simulink library "roblocks"  (R2019a)
settings: Solver=ode45  StartTime=0.0  StopTime=10  RelTol=1e-3  EnableMultiTasking=on
values from neighbouring files (symbols this model uses):
  q = 1    [quadrotor_plot.m]
undefined symbols (not defined in the file or in its folder): a, angdiff, camera, cinertia, cond, delta2tr, eul2tr, fkine, gravload, inertia, jacob0, jacobe, numcols, P, p560, purepursuit, qd, qdd, qz, rne, robot, rpy2tr, tr2delta, tr2eul, tr2rpy, transl, trnorm, trotz, v_max
(part 1 of 2)
settings Model: Creator=n6334687  LastModifiedBy=corkep
settings DataIOCC: LimitDataPoints=on  SaveFormat=Array  SignalLoggingSaveFormat=ModelDataLogs  ReturnWorkspaceOutputs=off
settings OptimizationCC: ExpressionDepthLimit=2147483647  LifeSpan=inf
settings DebuggingCC: UnderspecifiedInitializationDetection=Classic  MergeDetectMultiDrivingBlocksExec=none  SolverPrmCheckMsg=warning  FcnCallInpInsideContextMsg=warning  AllowSymbolicDim=off  StateNameClashWarn=warning  PregeneratedLibrarySubsystemCodeDiagnostic=none  SFUnexpectedBacktrackingDiag=warning  SFNoUnconditionalDefaultTransitionDiag=warning  SFExecutionAtInitializationDiag=none  ArithmeticOperatorsInVariantConditions=warning
settings HardwareCC: ProdBitPerPointer=32  ProdBitPerSizeT=32  ProdBitPerPtrDiffT=32  ProdLargestAtomicFloat=None  ProdIntDivRoundTo=Undefined  ProdEndianess=Unspecified  ProdWordSize=32  ProdHWDeviceType=32-bit Generic
settings ModelReferenceCC: PropagateSignalLabelsOutOfModel=off
settings SFSimCC: SimUseLocalCustomCode=off
settings RTWCC: RTWUseLocalCustomCode=off
settings CodeAppCC: StateflowObjectComments=on
settings GRTTargetCC: TargetLangStandard=C89/C90 (ANSI)  GeneratePreprocessorConditionals=Disable all  CombineOutputUpdateFcns=off  GRTInterface=on
settings ConfigComp: CovMetricSettings=dw  CovHtmlReporting=on  CovSaveCumulativeToWorkspaceVar=on  CovSaveSingleToWorkspaceVar=on  CovExternalEMLEnable=off  CovSFcnEnable=off

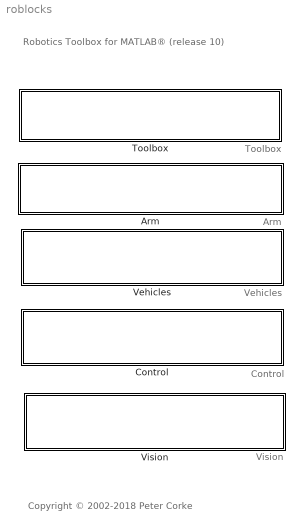
== system roblocks ==
  note: Vision
  note: Control
  note: Vehicles
  note: Arm
  note: Toolbox
  note: Robotics Toolbox for MATLAB®
      | (release 10)
  note: Copyright © 2002-2018 Peter Corke
  Arm : Subsystem
      mask Display: disp('Robot arms')
  Control : Subsystem
      mask Display: disp('Control')
  Toolbox : Subsystem
      mask Display: disp('Toolbox functions')
  Vehicles : Subsystem
      mask Display: disp('Vehicles: wheeled, flying')
  Vision : Subsystem
      mask Display: disp('Vision')

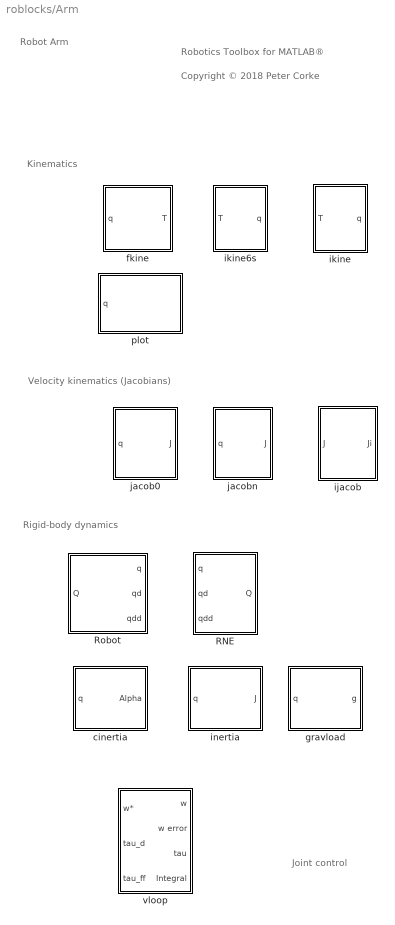
== system roblocks/Arm ==
  note: Robot
      | Arm
  note: Kinematics
  note: Velocity kinematics (Jacobians)
  note: Rigid-body dynamics
  note: Joint control
  note: Copyright © 2018 Peter Corke
  note: Robotics Toolbox for MATLAB®
  RNE : Subsystem  mask{robot=robot, grav=[0 0 9.81]}
      mask prompts: robot "Robot object"; grav "Gravity"
      mask help: Rigid-body inverse dynamics.
      mask init:
      | if isa(robot, 'SerialLink')
      |     n = robot.n
      |     rname = robot.name;
      | else
      |     n = 0;
      |     rname = '';
      | end
      mask Help:
      | Given a robot dynamic model and joint angle, rate and acceleration
      | determine the required joint torque.
      | 
      | <b>Parameters::</b>
      | 
      | robot (SerialLink) a dynamic model of an N-link serial link manipulator
      | gravity (1x3)  IGNORED Gravitational acceleration in world frame [m/s2]
      | 
      | <b>Inputs::</b>
      | 
      | q (1xN) joint coordinates
      | qd (1xN) joint coordinate velocity
      | qdd (1xN) joint coordinate acceleration
      | 
      | 
      | <b>Outputs::</b>
      | 
      | Q (1xN) the generalized joint force (torque or force) required to achieve
      | the motion state (q, qd, qdd).
      | 
      | <b>Notes::</b>
      | 
      | - Required for computed and inverse torque control schemes.
      | - The gravity parameter is ignored.
      | - Implemented using the recursive Newton-Euler scheme (RNE).
      | - A wrapper for the Toolbox method rne().
      mask Display:
      | port_label('output', 1, 'Q')
      | port_label('input', 1, 'q')
      | port_label('input', 2, 'qd')
      | port_label('input', 3, 'qdd')
      | text(0.9, 0.9,  rname, 'horizontalAlignment', 'right')
  Robot : Subsystem  mask{robot=robot, q0=[0 0 0 0 0 0]}
      mask prompts: robot "Robot object"; q0 "Initial state"
      mask help: Rigid-body dynamic model of robot.
      mask init:
      | if isa(robot, 'SerialLink')
      |     rname = robot.name;
      |     %fprintf('**robot name is %s\n', rname);
      | else
      |     rname = '';
      |     n = 0
      | end
      mask Help:
      | Simulates the forward (direct) rigid-body dynamics of the robot described
      | by the given robot object.  For given applied joint torque/force it computes
      | the instaneous joint coordinates, velocities and acclerations.
      | 
      | 
      | <b>Parameters::</b>
      | 
      | robot (SerialLink) a dynamic model of an N-link serial link manipulator
      | q0 (1xN)  Initial joint coordinates
      | 
      | <b>Inputs::</b>
      | 
      | Q (1xN) the generalized joint force (torque or force) required to achieve
      | the motion state (q, qd, qdd).
      | 
      | <b>Outputs::</b>
      | 
      | q (1xN) joint coordinates
      | qd (1xN) joint coordinate velocity
      | qdd (1xN) joint coordinate acceleration
      | 
      | 
      | <b>Notes::</b>
      | 
      | - Required to simulate robot rigid body motion.
      | - Implemented using the recursive Newton-Euler scheme (RNE).
      | - A wrapper for the Toolbox method accel() which in turn depends on the
      |   method rne().
      mask Display:
      | port_label('input', 1, 'Q')
      | port_label('output', 1, 'q')
      | port_label('output', 2, 'qd')
      | port_label('output', 3, 'qdd')
      | text(0.1, 0.9,  rname, 'horizontalAlignment', 'left')
  cinertia : Subsystem  mask{robot=0}
  fkine : Subsystem  mask{robot=robot}
      mask prompts: robot "Robot object"
      mask help: Robot forward kinematics.
      mask Help:
      | Compute homogeneous transform for robot end-effector given joint coordinates
      | 
      | 
      | <b>Parameters::</b>
      | 
      | Robot (SerialLink class)  The N-axis robot object for computing forward kinematics.
      | 
      | <b>Inputs::</b>
      | 
      | q (1xN) joint coordinates
      | 
      | <b>Outputs::</b>
      | 
      | T (4x4) the pose of the end effector as a homogeneous transformation
      | 
      | <b>Notes::</b>
      | 
      | - A wrapper for the Toolbox method fkine().
      mask Display:
      | port_label('input', 1, 'q')
      | port_label('output', 1, 'T')
      | if ~isempty(robot)
      |     text(0.5, 0.2, robot.name,  'horizontalAlignment', 'center')
      | end
  gravload : Subsystem  mask{robot=0}
  ijacob : Subsystem
      mask help: Inverse Jacobian
      mask Help:
      | Inverse of Jacobian matrix which maps spatial velocity to joint coordinate
      | rates.
      | 
      | 
      | <b>Inputs::</b>
      | 
      | J (6x6) the Jacobian matrix
      | 
      | <b>Outputs::</b>
      | 
      | Ji (6x6) the inverse Jacobian matrix
      | 
      | <b>Notes::</b>
      | 
      | - A wrapper for the MATLAB function inv().
      | - Only valid for square Jacobians (6-axis robots)
      mask Display:
      | text(0.4, 0.7, '\bf\fontsize{16}J', 'texmode', 'on', 'verticalAlignment', 'top', 'horizontalAlignment', 'left')
      | text(0.6, 0.65, '\fontsize{10}-1', 'texmode', 'on','verticalAlignment', 'bottom', 'horizontalAlignment', 'left')
      | port_label('input', 1, 'J');
      | port_label('output', 1, 'Ji')
  ikine : Subsystem  mask{robot=p560, q0=qz, M=[1 1 1 1 1 1], pinv=off, options={}}
      mask prompts: robot "Robot object"; q0 "Initial q"; M "Mask vector"; pinv "Pseudo-inverse (pinv)"; options "Options (cell array)"
      mask help: Generalized numerical inverse kinematics
      mask init:
      | opt = options;
      | if pinv
      |     opt = [opt 'pinv'];
      | end
      | disp(opt)
      mask Help:
      | Compute joint coordinates for robot given end-effector pose.
      | 
      | 
      | <b>Parameters::</b>
      | 
      | Robot (SerialLink class)  The N-axis robot object for computing forward kinematics.
      | Initial q  (1xN)          Initial joint coordinates for solution
      | Mask vector (1x6)         Mask vector for underactuated manipulators.
      | Pseudo inverse (logical)  Enable option 'pinv'
      | Options                   Option value list to be passed to ikine()
      | 
      | <b>Inputs::</b>
      | 
      | T (4x4) the pose of the end effector as a homogeneous transformation
      | 
      | 
      | <b>Outputs::</b>
      | 
      | q (1xN) joint coordinates
      | 
      | <b>Notes::</b>
      | 
      | - A wrapper for the Toolbox method ikine().
  ikine6s : Subsystem  mask{robot=p560, conf='luf'}
      mask prompts: robot "Robot object"; conf "Configuration string"
      mask help: Inverse kinematics for 6-axis spherical robot
      mask Help:
      | Compute joint coordinates for robot given end-effector pose.
      | 
      | 
      | <b>Parameters::</b>
      | 
      | Robot (SerialLink class)  The N-axis robot object for computing forward kinematics.
      | Configuration             Configuration string comprised of 'lrudnf'
      | 
      | <b>Inputs::</b>
      | 
      | T (4x4) the pose of the end effector as a homogeneous transformation
      | 
      | 
      | <b>Outputs::</b>
      | 
      | q (1xN) joint coordinates
      | 
      | <b>Notes::</b>
      | 
      | - A wrapper for the Toolbox method ikine6s().
  inertia : Subsystem  mask{robot=0}
  "jacob0 " : Subsystem  mask{robot=robot}
      mask prompts: robot "Robot object"
      mask help: Robot Jacobian in world coordinates
      mask init:
      | if ~isempty(robot)
      |     n=robot.n;
      | end
      mask Help:
      | Jacobian matrix relating joint coordinate rates to end-effector spatial
      | velocity expressed in the world frame.
      | 
      | <b>Parameters::</b>
      | 
      | Robot (SerialLink class)  The N-axis robot object for which the Jacobian is
      |                           computed.
      | 
      | <b>Inputs::</b>
      | 
      | q (1xN) joint coordinates
      | 
      | <b>Outputs::</b>
      | 
      | J (6xN) the Jacobian matrix
      | 
      | <b>Notes::</b>
      | 
      | - A wrapper for the Toolbox method jacob0().
      mask Display:
      | text(0.4, 0.7, '\bf\fontsize{16}J', 'texmode', 'on', 'verticalAlignment', 'top', 'horizontalAlignment', 'left')
      | text(0.45, 0.65, '\fontsize{10}0', 'texmode', 'on','verticalAlignment', 'bottom', 'horizontalAlignment', 'right')
      | if ~isempty(robot)
      |     text(0.5, 0.2, robot.name,  'horizontalAlignment', 'center')
      | end
      | port_label('input', 1, 'q')
      | port_label('output', 1, 'J')
  jacobn : Subsystem  mask{robot=robot}
      mask prompts: robot "Robot object"
      mask help: Robot Jacobian in end-effector coordinates
      mask init:
      | n=robot.n;
      mask Help:
      | Jacobian matrix relating joint coordinate rates to end-effector spatial
      | velocity expressed in the end-effector frame.
      | 
      | <b>Parameters::</b>
      | 
      | Robot (SerialLink class)  The N-axis robot object for which the Jacobian is
      |                           computed.
      | 
      | <b>Inputs::</b>
      | 
      | q (1xN) joint coordinates
      | 
      | <b>Outputs::</b>
      | 
      | J (6xN) the Jacobian matrix
      | 
      | <b>Notes::</b>
      | 
      | - A wrapper for the Toolbox method jacobn().
      mask Display:
      | text(0.4, 0.7, '\bf\fontsize{16}J', 'texmode', 'on', 'verticalAlignment', 'top', 'horizontalAlignment', 'left')
      | text(0.45, 0.65, '\fontsize{10}N', 'texmode', 'on','verticalAlignment', 'bottom', 'horizontalAlignment', 'right')
      | if ~isempty(robot)
      |     text(0.5, 0.2, robot.name,  'horizontalAlignment', 'center')
      | end
      | port_label('input', 1, 'q')
      | port_label('output', 1, 'J')
  plot : Subsystem  mask{robot=p560, fps=5, holdplot=on}
      mask prompts: robot "Robot object"; fps "Update rate (fps)"; holdplot "Hold"
      mask help: Graphical robot display.
      mask Help:
      | This block graphically displays the passed SerialLink class object.
      | 
      | A new figure is created and the robot is animated (using SerialLink.plot)
      | to a pose specified by the joint coordinate vector input to the block whose
      | width must match the number of robot joints.
      | 
      | If the Hold checkbox is ticked then a "hold" command is issued at initialization
      | time allowing multiple robots to be displayed in the one plot.
      mask Display:
      | port_label('input', 1, 'q')
      | if ~isempty(robot)
      |     text(0.5, 0.2, robot.name,  'horizontalAlignment', 'center')
      | end
  vloop : Subsystem  mask{J=372e-6, B=817e-6, Km=0.228, tau_max=0.9, Kv=1, Ki=0, T=0.001}
      mask prompts: J "Inertia (J)"; B "Viscous friction coefficient (B)"; Km "Motor torque constant"; tau_max "Torque limit (tau_max)"; Kv "Proportional gain (Kv)"; Ki "Integral gain (Ki)"; T "Sample interval (T)"

== system roblocks/Control ==
  note: Robotics Toolbox for MATLAB®
  note: Copyright © 2018 Peter Corke
  note: Control
  note: Motor control
  vloop_voltage : Subsystem  mask{J=372e-6, B=817e-6, Km=0.228, tau_max=20, Rm=0.1, Lm=0.1, Ka=10, Kv=1, Ki=1, T=0.001}
      mask prompts: J "Inertia (K)"; B "Viscous friction coefficient (B)"; Km "Motor torque constant"; tau_max "Voltage limit (tau_max)"; Rm "Motor resistance (Rm)"; Lm "Motor inductance (Lm)"; Ka "Amplifier gain (Ka)"; Kv "Proportional gain (Kv)"; Ki "Integral gain (Ki)"; T "Sample interval (T)"

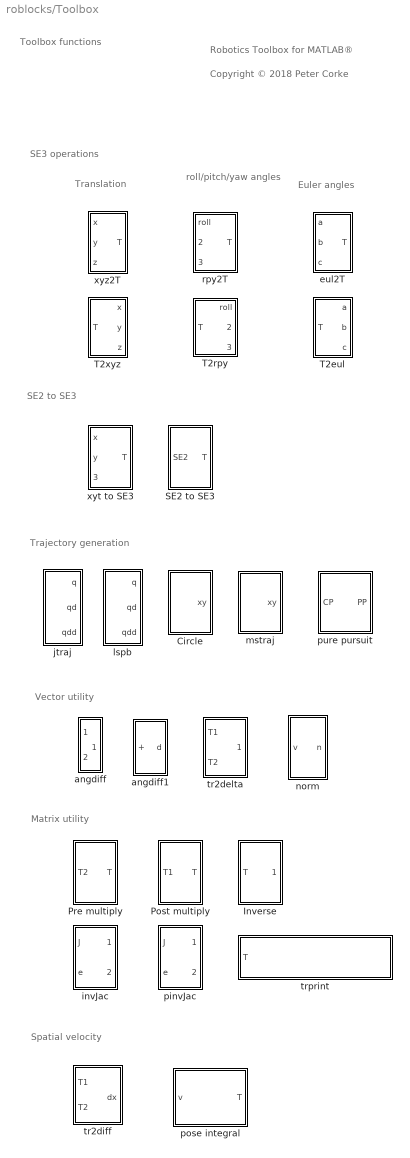
== system roblocks/Toolbox ==
  note: SE2 to SE3
  note: Vector utility
  note: Matrix utility
  note: Trajectory generation
  note: Spatial velocity
  note: SE3 operations
  note: Robotics Toolbox for MATLAB®
  note: Translation
  note: roll/pitch/yaw
      | angles
  note: Euler angles
  note: Toolbox
      | functions
  note: Copyright © 2018 Peter Corke
  Circle : Subsystem  mask{radius=1, freq=0.2}
      mask prompts: freq "Frequency (rev/s)"
      mask help: Generate circular trajectory
      mask Help:
      | Generate circular trajectory in the xy-plane and centred at the origin.
      | 
      | <b>Parameters::</b>
      | 
      | radius   The radius of the circle [m]
      | freq     The frequency of motion [rev/s]
      | 
      | <b>Output::</b>
      | 
      | xy (1x2) a vector of xy-coordinates at the current simulation time step.
      | 
      | <b>Notes::</b>
      | - Motion is at constant velocity around the circle, there is an infinite
      |   initial acceleration.
      | - The motion continues for the whole simulation.
  Inverse : Subsystem
      mask help: Inverse of homogeneous transformation
      mask Help:
      | Inverse of homogeneous transformation
      | 
      | 
      | <b>Inputs::</b>
      | 
      | T (4x4) Incoming homogeneous transform
      | 
      | <b>Outputs::</b>
      | 
      | invT (4x4) Outgoing homogeneous transformation T^(-1)
      | 
      | <b>Notes::</b>
      | - Efficient implementation that uses transpose of rotation submatrix.
  Post multiply : Subsystem  mask{T2=0}
      mask prompts: T2 "TP"
      mask help: Post-multiply incoming transform by a constant transformation
      mask Help:
      | Post-multiply homogeneous transform signal by a constant transform.
      | 
      | <b>Parameters::</b>
      | 
      | TP (4x4)  The transform to post-multiply by
      | 
      | <b>Inputs::</b>
      | 
      | T1 (4x4) Incoming homogeneous transform
      | 
      | <b>Outputs::</b>
      | 
      | T (4x4) Outgoing homogeneous transformation is T1*TP
  Pre multiply : Subsystem  mask{T=0}
      mask prompts: T "T1"
      mask help: Pre-multiply homogeneous transform by constant transform.
      mask Help:
      | Pre-multiply homogeneous transform signal by a constant transform.
      | 
      | <b>Parameters::</b>
      | 
      | TP (4x4)  The transform to pre-multiply by
      | 
      | <b>Inputs::</b>
      | 
      | T2 (4x4) Incoming homogeneous transform
      | 
      | <b>Outputs::</b>
      | 
      | T (4x4) Outgoing homogeneous transformation is TP*T2
  SE2 to SE3 : Subsystem
      mask Display:
      | port_label('input', 1, 'xyt')
      | port_label('output', 1, 'T')
  T2eul : Subsystem  mask{degrees=off}
      mask prompts: degrees "Use degrees"
      mask help: Convert transform to Euler angles.
      mask init:
      | if degrees
      |     args = {'deg'};
      | else
      |     args = {};
      | end
      mask Help:
      | Convert homogeneous transformation to Euler angles.
      | 
      | 
      | <b>Inputs::</b>
      | 
      | T (4x4) the attitude as a homogeneous transformation
      | 
      | <b>Outputs::</b>
      | 
      | phi (1x1) first Euler angle [rad]
      | theta (1x1) second Euler angle [rad]
      | psi (1x1) third Euler angle [rad]
      | 
      | <b>Notes::</b>
      | 
      | - Axis rotation order is z-y-z (aerospace convention).
      | - Wrapper for the Toolbox function tr2eul().
      mask Display:
      | port_label('output', 1, '\phi', 'texmode', 'on')
      | port_label('output', 2, '\theta', 'texmode', 'on')
      | port_label('output', 3, '\psi', 'texmode', 'on')
      | port_label('input', 1, 'T')
  T2rpy : Subsystem  mask(Transform to roll-pitch-yaw angles){sequence=ZYX, degrees=off}
      mask prompts: sequence "Angle sequence (yaw, pitch, roll)"; degrees "Use degrees"
      mask help:
      | Convert transform to roll/pitch/yaw angles.
      |
      | yaw about first axis in sequence [-pi pi)
      | pitch about second axis  in sequence [-pi/2 pi/2)
      | roll about third axis  in sequence [-pi pi)
      |
      | Angles are in radians by default.
      mask init:
      | sequences = {'zyx', 'xyz', 'yxz'};
      | args = {sequences{sequence}};
      | if degrees
      |     args = [args 'deg'];
      | end
      mask Help:
      | Convert homogeneous transformation to roll/pitch/yaw angles.
      | 
      | Rotate about the axes given in the sequence:
      | 
      | <ul>
      | <li>roll (1x1) roll angle &isin; [-&pi; &pi;)</li>
      | <li>pitch (1x1) pitch angle &isin; [-&pi;/2 &pi;/2)</li>
      | <li>yaw (1x1) yaw angle &isin; [-&pi; &pi;)</li>
      | </ul>
      | 
      | <h2>Inputs::</h2>
      | 
      | T (4x4) the pose as a homogeneous transformation
      | 
      | <h2>Outputs::</h2>
      | 
      | <ul>
      | <li>roll (1x1) roll angle </li>
      | <li>pitch (1x1) pitch angle </li>
      | <li>yaw (1x1) yaw angle </li>
      | </ul>
      | 
      | <h2>Notes::</h2>
      | 
      | - Axis rotation order is x-y-z (aerospace convention).
      | - Wrapper for the Toolbox function tr2rpy().
      mask TypeOptions sequence: ZYX | XYZ | YXZ
  T2xyz : Subsystem
      mask help: Convert transform to xyz scalars
      mask Help:
      | Convert homogeneous transformation to position scalars.
      | 
      | 
      | <b>Inputs::</b>
      | 
      | T (4x4) a translation represented as a homogeneous transformation
      | 
      | <b>Outputs::</b>
      | 
      | x (1x1) x-coordinate
      | y (1x1) y-coordinate
      | z (1x1) z-coordinate
      | 
      | <b>Notes::</b>
      | 
      | - A wrapper for the Toolbox function transl().
  angdiff : Subsystem
      mask help: Difference of angles wrapped into the range -pi to +pi
      mask Help:
      | A difference block for angles and the result is guaranteed to be in the
      | interval [-&pi;pi +&pi;).
      | 
      | <b>Notes::</b>
      | - Is a wrapper for the Toolbox function angdiff.
  angdiff1 : Subsystem
      mask help: Wrap angle to range -pi to +pi
      mask Help:
      | A difference block for angles and the result is guaranteed to be in the
      | interval [-&pi;pi +&pi;).
      | 
      | <b>Notes::</b>
      | - Is a wrapper for the Toolbox function angdiff.
      mask Display:
      | port_label('input', 1, '\theta', 'texmode', 'on')
      | port_label('output', 1, '\theta''', 'texmode', 'on')
  eul2T : Subsystem  mask{degrees=off}
      mask prompts: degrees "Use degrees"
      mask help: Convert Euler angles to transform.
      mask init:
      | if degrees
      |     args = {'deg'};
      | else
      |     args = {};
      | end
      mask Help:
      | Convert Euler angles to homogeneous transformation.
      | 
      | 
      | <b>Inputs::</b>
      | 
      | phi (1x1) first Euler angle [rad]
      | theta (1x1) second Euler angle [rad]
      | psi (1x1) third Euler angle [rad]
      | 
      | 
      | <b>Outputs::</b>
      | 
      | T (4x4) the attitude as a homogeneous transformation
      | 
      | <b>Notes::</b>
      | 
      | - Axis rotation order is z-y-z (aerospace convention).
      | - Wrapper for the Toolbox function eul2tr().
      mask Display:
      | port_label('input', 1, '\phi', 'texmode', 'on')
      | port_label('input', 2, '\theta', 'texmode', 'on')
      | port_label('input', 3, '\psi', 'texmode', 'on')
      | port_label('output', 1, 'T')
  invJac : Subsystem
      mask help: Inverse image Jacobian
      mask Help:
      | Computes camera velocity based on the inverse image Jacobian and image
      | plane error.
      | 
      | 
      | <b>Inputs::</b>
      | 
      | J (6x6) the image Jacobian matrix
      | e (6x1) the image plane error (du1, dv1, du2, dv2, ...)
      | 
      | <b>Outputs::</b>
      | 
      | vdot (1x6) the required camera spatial velocity
      | cond (1x1) the condition of the image Jacobian
      | 
      | <b>Notes::</b>
      | 
      | - A wrapper for the MATLAB function inv().
      | - Only valid for square Jacobians (3 image points)
  jtraj : Subsystem  mask{q0=[0 0 0 0 0 0], qf=[pi/4 pi/2 -pi/2 0 0 0], tmax=10, ts=0.02}
      mask prompts: tmax "tmax (s)"; ts "ts (s)"
      mask help: Joint interpolated trajectory.
      mask init:
      | n = length(q0);
      | if length(q0) ~= length(qf) ,
      |  error('q0 and qf must be same length')
      | end
      | t=[0:100]'/100*tmax;
      | [q,qd,qdd] = jtraj(q0, qf, t);
      mask Help:
      | Generate quintic polynomial to move from initial to final joint angles as specified.  Initial and final velocity are assumed to be zero.
      | 
      | <b>Parameters::</b>
      | 
      | q0 (1xN) initial joint coordinates
      | qf (1xN) final joint coordinates
      | tmax (1x1) the time for the trajectory to complete
      | 
      | Initial and final velocity are assumed to be zero.
      | 
      | <b>Outputs::</b>
      | 
      | q (1xN) vector of joint coordinates at current simulation time
      | qd (1xN) vector of joint coordinate velocity at current simulation time
      | qdd (1xN) vector of joint coordinate acceleration at current simulation time
      | 
      | <b>Notes::</b>
      | 
      | - If simulation time exceeds tmax then q is clipped to qf.
      | - A wrapper on the Toolbox function jtraj.
      | - The piecewise constant output of jtraj is interpolated to the current
      |   simulation time.
      mask Display:
      | port_label('output', 1, 'q')
      | port_label('output', 2, 'qd')
      | port_label('output', 3, 'qdd')
  lspb : Subsystem  mask{q0=0, qf=0, tmax=0}
      mask help: Scalar trajectory.
      mask init:
      | n = length(q0);
      | if length(q0) ~= length(qf) ,
      |  error('q0 and qf must be same length')
      | end
      | t=[0:1000]'/1000*tmax;
      | [q,qd,qdd] = lspb(q0, qf, t);
      mask Help:
      | Generate linear segment with polynomial blend to move from initial to final
      |  joint angles as specified.
      | 
      | <b>Parameters::</b>
      | 
      | q0 (1x1) initial joint coordinate
      | qf (1x1) final joint coordinate
      | tmax (1x1) the time for the trajectory to complete
      | 
      | Initial and final velocity are assumed to be zero.
      | 
      | <b>Outputs::</b>
      | 
      | q (1x1) joint coordinates at current simulation time
      | qd (1x1) joint coordinate velocity at current simulation time
      | qdd (1xN) joint coordinate acceleration at current simulation time
      | 
      | <b>Notes::</b>
      | 
      | - If simulation time exceeds tmax then q is clipped to qf.
      | - A wrapper on the Toolbox function lspb.
      | - The piecewise constant output of jtraj is interpolated to the current simulation time.
  mstraj : Subsystem  mask(Trajectory generator){path=|, vaxis=[2.5 2.5], tseg=[], dt=0.1, tacc=0, setsimtime=on}
      mask path=|
      | [  10 10;
      |   10 60;
      |   80 80;
      |   50 10 ]
      mask prompts: vaxis "Axis velocities"; tseg "Segment times"; dt "Sample interval"; tacc "Acceleration time"; setsimtime "Set Simulink simulation time"
      mask help: Generate an n-dimensional trajectory using the Toolbox function mstraj.
      mask init:
      | robot_traj = mstraj(path(2:end,:), vaxis, tseg, path(1,:), dt, tacc);
      | total_time = size(robot_traj,1)*dt;
      | if setsimtime
      |     set_param(gcs, 'StopTime', num2str(total_time));
      | end
      mask Help:
      | The trajectory requires a number of parameters
      | 
      | Path: an MxN matrix that defines a path with M points (start, intermediate, goal) and each point is defined by an N-dimensional vector.
      | 
      | Axis velocities: a 1xM vector that specifies the maximum speed of each motion for each dimension.
      | 
      | Segment times: a 1x(N-1) vector of times to execute each motion segment.
      | 
      | Sample time: a scalar sampling time, the trajectory is computed at discrete times with this separation.
      | 
      | Acceleration time: a scalar giving the period of acceleration at each waypoint, as the motion accelerates from one segment to the next.  Can be zero.
      | 
      | This block sets the Simulink simulation time to the length of the trajectory.
      mask Display: plot(path(:,1), path(:,2))
  norm : Subsystem
      mask Display:
      | port_label('output', 1, '|v|', 'texmode', 'on')
      | port_label('input', 1, 'v')
  pinvJac : Subsystem
      mask help: Inverse image Jacobian
      mask Help:
      | Computes camera velocity based on the pseudo-inverse of the image Jacobian
      | and image plane error for more than 3 points.
      | 
      | 
      | <b>Inputs::</b>
      | 
      | J (2Nx6) the image Jacobian matrix
      | e (2Nx1) the image plane error (du1, dv1, du2, dv2, ...)
      | 
      | <b>Outputs::</b>
      | 
      | vdot (1x6) the required camera spatial velocity
      | cond (1x1) the condition of the image Jacobian
      | 
      | <b>Notes::</b>
      | 
      | - A wrapper for the MATLAB function pinv().
      | - Valid for non-square Jacobians (>=3 image points)
  pose integral : Subsystem  mask{T0=transl(0,0,1)*trotz(1.5), dt=0.02}
      mask prompts: T0 "Initial pose (hom transform)"; dt "Sample interval (s)"
      mask help: Integrate spatial velocity
      mask Help:
      | Integrate spatial velocity to update pose represented as a homogeneous
      | transformation.
      | 
      | <b>Parameters::</b>
      | 
      | T0 (4x4)  The initial pose
      | dt (1x1)  The sample interval [s]
      | 
      | <b>Inputs::</b>
      | 
      | v (1x6) spatial velocity (xd yd zd wx wy wz)
      | 
      | <b>Outputs::</b>
      | 
      | T (4x4) the integrated pose as a homogeneous transformation
      | 
      | <b>Notes::</b>
      | 
      | - Contains a unit delay of dt
      | - The transform is kept normalized using trnorm().
  pure pursuit : Subsystem  mask(Trajectory generator){path=|, vaxis=[2.5 2.5], tseg=[], dt=0.1, tacc=0, R=5}
      mask path=|
      | [  10 10;
      |   10 60;
      |   80 80;
      |   50 10 ]
      mask prompts: vaxis "Axis velocities"; tseg "Segment times"; dt "Sample interval"; tacc "Acceleration time"; R "Look ahead distance"
      mask help: Generate an n-dimensional trajectory using the Toolbox function mstraj.
      mask init:
      | robot_traj = mstraj(path(2:end,:), vaxis, tseg, path(1,:), dt, tacc);
      | total_time = size(robot_traj,1)*dt;
      mask Help:
      | The trajectory requires a number of parameters
      | 
      | Path: an MxN matrix that defines a path with M points (start, intermediate, goal) and each point is defined by an N-dimensional vector.
      | 
      | Axis velocities: a 1xM vector that specifies the maximum speed of each motion for each dimension.
      | 
      | Segment times: a 1x(N-1) vector of times to execute each motion segment.
      | 
      | Sample time: a scalar sampling time, the trajectory is computed at discrete times with this separation.
      | 
      | Acceleration time: a scalar giving the period of acceleration at each waypoint, as the motion accelerates from one segment to the next.  Can be zero.
      | 
      | This block sets the Simulink simulation time to the length of the trajectory.
      mask Display: plot(path(:,1), path(:,2))
  rpy2T : Subsystem  mask(Roll-pitch-yaw angles to transform){sequence=ZYX, degrees=off}
      mask prompts: sequence "Angle sequence (yaw, pitch, roll)"; degrees "Use degrees"
      mask help:
      | Convert roll/pitch/yaw angles to transform.  Rotate about the axes given in the sequence:
      |
      | yaw about first axis in sequence
      | pitch about second axis  in sequence
      | roll about third axis  in sequence
      |
      | Angles are in radians by default.
      mask init:
      | sequences = {'zyx', 'xyz', 'yxz'};
      | args = {sequences{sequence}};
      | if degrees
      |     args = [args 'deg'];
      | end
      mask Help:
      | Convert roll/pitch/yaw angles to homogeneous transformation.
      | 
      | Rotate about the axes given in the sequence:
      | <ul>
      | <li>yaw about first axis in sequence</li>
      | <li>pitch about second axis  in sequence</li>
      | <li>roll about third axis  in sequence</li>
      | </ul>
      | 
      | <h2>Inputs::</h2>
      | 
      | <ul>
      | <li>yaw about first axis in sequence </li>
      | <li>pitch about second axis  in sequence</li>
      | <li>roll about third axis  in sequence</li>
      | </ul>
      | 
      | <h2>Outputs::</h2>
      | 
      | T (4x4) the pose as a homogeneous transformation
      | 
      | <h2>Notes::</h2>
      | 
      | - Wrapper for the Toolbox function rpy2tr().
      mask TypeOptions sequence: ZYX | XYZ | YXZ
  tr2delta : Subsystem
      mask help: Convert transform to spatial displacement (d, theta).
      mask Help:
      | Compute the spatial displacement T1-T2 (as a 6-vector) between two poses given as
      | homogeneous transformations.
      | 
      | <b>Inputs::</b>
      | 
      | T1 (4x4) pose as a homogeneous transformation
      | T2 (4x4) pose as a homogeneous transformation
      | 
      | <b>Outputs::</b>
      | 
      | dx (1x6) the spatial displacement from T2 to T1 (dx dy dz dwx dwy dwz)
      | 
      | <b>Notes::</b>
      | 
      | - delta is the integral of a spatial velocity over time.
      | - A wrapper for the Toolbox function tr2delta().
      mask Display:
      | port_label('input', 1, 'T_1', 'texmode', 'on')
      | port_label('input', 2, 'T_2', 'texmode', 'on')
      | port_label('output', 1, '\delta', 'texmode', 'on')
  tr2diff : Subsystem  mask{robot=robot}
      mask prompts: robot "Robot object"
      mask help: Compute differential motion
      mask Help:
      | Compute the differential motion (as a 6-vector) between two poses given as
      | homogeneous transformations.
      | 
      | <b>Inputs::</b>
      | 
      | T1 (4x4) initial pose as a homogeneous transformation
      | T2 (4x4) final pose as a homogeneous transformation
      | 
      | <b>Outputs::</b>
      | 
      | dx (1x6) the differential motion (dx dy dz dwx dwy dwz)
      | 
      | <b>Notes::</b>
      | 
      | - Only valid for infinitessimal displacements.
      | - dx is the integral of a spatial velocity over time.
      | - A wrapper for the Toolbox function tr2delta().
      mask Display:
      | port_label('input', 1, 'T1')
      | port_label('input', 2, 'T2')
      | port_label('output', 1, 'dx')
  trprint : Subsystem  mask{options={'bingo'}}
      mask prompts: options "Options (cell array)"
      mask Display: disp('t = (0,0,0), RPY = (0,0,0) deg');
  xyt to SE3 : Subsystem
      mask Display:
      | port_label('input', 1, 'x')
      | port_label('input', 2, 'y')
      | port_label('input', 3, '\theta', 'texmode', 'on')
      | port_label('output', 1, 'T')
  xyz2T : Subsystem
      mask help: Convert xyz scalars to transform.
      mask Help:
      | Convert position scalars to a homogeneous transformation.
      | 
      | 
      | <b>Inputs::</b>
      | 
      | x (1x1) x-coordinate
      | y (1x1) y-coordinate
      | z (1x1) z-coordinate
      | 
      | 
      | <b>Outputs::</b>
      | 
      | T (4x4) a translation represented as a homogeneous transformation
      | 
      | <b>Notes::</b>
      | 
      | - A wrapper for the Toolbox function transl().

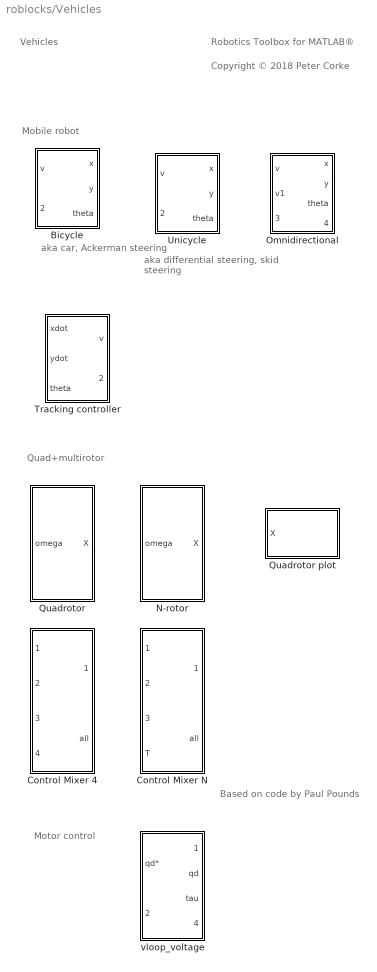
== system roblocks/Vehicles ==
  note: Motor control
  note: Quad+multirotor
  note: aka differential steering, skid steering
  note: aka car, Ackerman steering
  note: Mobile robot
  note: Based on code by Paul Pounds
  note: Vehicles
  note: Robotics Toolbox for MATLAB®
  note: Copyright © 2018 Peter Corke
  Bicycle : Subsystem  mask{vlim=1, accel=Inf, alim=2, steer_rate=Inf, L=1, x0=[0, 0, 0]}
      mask prompts: vlim "Velocity limit (m/s)"; accel "Acceleration limit (m/s2)"; alim "Steering angle limit (rad)"; steer_rate "Steering rate limit (rad/s)"; L "Wheel base"; x0 "Initial state (x, y, theta)"
      mask help: Kino-dynamic model of bicycle vehicle
      mask Help:
      | Kino-dynamic model of bicycle vehicle, also known as Ackermann vehicle
      | model.
      | 
      | <b>Parameters::</b>
      | 
      | Acceleration (1x1)   Vehicle acceleration limit [m/s2]
      | Velocity limit (1x1)  Vehicle speed limit [m/s]
      | Steering limits (1x1) Steering angle limit [rad]
      | Initial state (1x3) Initial state (x, y, theta)
      | Handbrake (1x1) Vehicle cannot move if non-zero
      | 
      | <b>Inputs::</b>
      | 
      | v (1x1) velocity demand [m/s]
      | gamma (1x1) steering angle [rad]
      | 
      | <b>Outputs::</b>
      | 
      | x (1x1) x-coordinate in world frame [m]
      | y (1x1) x-coordinate in world frame [m]
      | theta (1x1) heading angle in world frame [rad]
      | 
      | 
      | <b>Notes::</b>
      | 
      | - Steering limit is symmetric between -limit and +limit
      | - Same dynamic model as the Toolbox class Vehicle.
      mask Display:
      | port_label('input', 1, 'v')
      | port_label('input', 2, '\gamma', 'texmode', 'on')
      | port_label('output', 1, 'x')
      | port_label('output', 2, 'y')
      | port_label('output', 3, '\theta', 'texmode', 'on')
  Control Mixer 4 : Subsystem  mask{quad=[], maxrot=0, minrot=0}
      mask prompts: quad "Quadrotor parameters"; maxrot "Maximum rotor speed (rad/s)"; minrot "Minimum rotor speed (rad/s)"
      mask help: Quadrotor control mixer
      mask Help:
      | Determine rotor speeds based on desired torques and thrust, and propellor model
      | 
      | <b>Inputs::</b>
      | tau<sub>x</sub> (1x1)    desired rolling torque [Nm]
      | 
      | tau<sub>y</sub> (1x1)    desired pitching torque [Nm]
      | tau<sub>z</sub> (1x1)    desired yawing torque [Nm]
      | T (1x1)          desired thrust [N]
      | 
      | <b>Outputs::</b>
      | 
      | w1 (1x1) angular velocity of rotor 1 [rad]
      | w2 (1x1) angular velocity of rotor 2 [rad]
      | w3 (1x1) angular velocity of rotor 3 [rad]
      | w4 (1x1) angular velocity of rotor 4 [rad]
      | 
      | <b>Notes::</b>
      | 
      | - Assumes the rotor labelling convention of RVC Fig 4.16.
      | - The quadrotor is underactuated and has only 4 inputs.
      mask Display:
      | port_label('output',1,'\varpi','texmode','on');
      | port_label('output',2,'\tau_a','texmode','on');
      | port_label('input',1,'\tau_x','texmode','on');
      | port_label('input',2,'\tau_y','texmode','on');
      | port_label('input',3,'\tau_z','texmode','on');
      | port_label('input',4,'T','texmode','on');
  Control Mixer N : Subsystem  mask{nrotors=4, wmax=1000, wmin=100}
      mask prompts: nrotors "Number of rotors (even)"; wmax "Maximum rotor speed"; wmin "Minimum rotor speed"
      mask help: Quadrotor control mixer
      mask Help:
      | Determine rotor speeds based on desired torques and thrust.
      | 
      | <b>Inputs::</b>
      | 
      | tau pitch (1x1)  desired pitching torque [Nm]
      | tau roll (1x1)   desired rolling torque [Nm]
      | tau yaw (1x1)    desired yawing torque [Nm]
      | T (1x1)          desired thrust [N]
      | 
      | <b>Outputs::</b>
      | 
      | w1 (1x1) angular velocity of rotor 1 [rad]
      | w2 (1x1) angular velocity of rotor 2 [rad]
      | w3 (1x1) angular velocity of rotor 3 [rad]
      | w4 (1x1) angular velocity of rotor 4 [rad]
      | 
      | <b>Notes::</b>
      | 
      | - Assumes the rotor labelling convention of RVC Fig 4.16.
      | - The quadrotor is underactuated and has only 4 inputs.
      mask Display:
      | port_label('output',1,'\varpi','texmode','on');
      | port_label('output',2,'\tau_a','texmode','on');
      | port_label('input',1,'\tau_x','texmode','on');
      | port_label('input',2,'\tau_y','texmode','on');
      | port_label('input',3,'\tau_z','texmode','on');
      | port_label('input',4,'T','texmode','on');
  N-rotor : Subsystem  mask{quad=[], x0=0, groundflag=on}
      mask prompts: quad "Quadrotor params"; x0 "Initial position [x y z]"; groundflag "Ground"
      mask help: Quadrotor dynamics
      mask Help:
      | Integrate spatial velocity to update pose represented as a homogeneous
      | transformation.
      | 
      | <b>Parameters::</b>
      | 
      | q (struct)  A structure containing quadrotor dynamics
      | 
      | The elements of q are:
      | 
      |  J         Flyer rotational inertia matrix (3x3)
      |  h         Height of rotors above CoG (1x1)
      |  d         Length of flyer arms (1x1)
      |  nb        Number of blades per rotor (1x1)
      |  r         Rotor radius (1x1)
      |  c         Blade chord (1x1)
      |  e         Flapping hinge offset (1x1)
      |  Mb        Rotor blade mass (1x1)
      |  Mc        Estimated hub clamp mass (1x1)
      |  ec        Blade root clamp displacement (1x1)
      |  Ib        Rotor blade rotational inertia (1x1)
      |  Ic        Estimated root clamp inertia (1x1)
      |  mb        Static blade moment (1x1)
      |  Ir        Total rotor inertia (1x1)
      |  Ct        Non-dim. thrust coefficient (1x1)
      |  Cq        Non-dim. torque coefficient (1x1)
      |  sigma     Rotor solidity ratio (1x1)
      |  thetat    Blade tip angle (1x1)
      |  theta0    Blade root angle (1x1)
      |  theta1    Blade twist angle (1x1)
      |  theta75   3/4 blade angle (1x1)
      |  thetai    Blade ideal root approximation (1x1)
      |  a         Lift slope gradient (1x1)
      |  A         Rotor disc area (1x1)
      |  gamma     Lock number (1x1)
      | 
      | 
      | <b>Inputs::</b>
      | 
      | w1 (1x1) angular velocity of rotor 1 [rad]
      | w2 (1x1) angular velocity of rotor 2 [rad]
      | w3 (1x1) angular velocity of rotor 3 [rad]
      | w4 (1x1) angular velocity of rotor 4 [rad]
      | 
      | <b>Outputs::</b>
      | 
      | X (1x12) state vector (x, y, z, thr, thp, thy, xd, yd, zd, thrd, thpd, thyd)
      | 
      | (x,y,z) is the position in the world frame [m]
      | (thr, thp, thy) the roll/pitch/yaw orientation in the world frame [rad]
      | (xd,yd,zd) is the velocity in the body frame [m]
      | (thrd,thpd,thyd) is the roll/pitch/yaw rates in the body frame [rad/s]
      | 
      | <b>Notes::</b>
      | 
      | - See also mdl_quadrotor which defines parameters for the ANU X4 flyer.
      mask Display:
      | port_label('input',1,'\varpi','texmode','on');
      | port_label('output',1,'X','texmode','on');
  Omnidirectional : Subsystem  mask{accel=1, vlim=1, alim=2, L=0, x0=[0, 0, 0], P=[1 1 -1 -1; 1 -1 -1 1], alpha=[1 -1 1 -1]*pi/4, R=0.1}
      mask prompts: accel "Acceleration"; vlim "Velocity limit"; alim "Steering limits"; L "Wheel base"; x0 "Initial state (x, y, theta)"; P "Wheel positions"; alpha "Roller angle"; R "Wheel radius"
      mask help: Kino-dynamic model of bicycle vehicle
      mask Help:
      | Kino-dynamic model of bicycle vehicle, also known as Ackermann vehicle
      | model.
      | 
      | <b>Parameters::</b>
      | 
      | Acceleration (1x1)   Vehicle acceleration limit [m/s2]
      | Velocity limit (1x1)  Vehicle speed limit [m/s]
      | Steering limits (1x1) Steering angle limit [rad]
      | Initial state (1x3) Initial state (x, y, theta)
      | Handbrake (1x1) Vehicle cannot move if non-zero
      | 
      | <b>Inputs::</b>
      | 
      | v (1x1) velocity demand [m/s]
      | gamma (1x1) steering angle [rad]
      | 
      | <b>Outputs::</b>
      | 
      | x (1x1) x-coordinate in world frame [m]
      | y (1x1) x-coordinate in world frame [m]
      | theta (1x1) heading angle in world frame [rad]
      | 
      | 
      | <b>Notes::</b>
      | 
      | - Steering limit is symmetric between -limit and +limit
      | - Same dynamic model as the Toolbox class Vehicle.
      mask Display:
      | port_label('input', 1, 'v_x', 'texmode', 'on')
      | port_label('input', 2, 'v_y', 'texmode', 'on')
      | port_label('input', 3, '\omega', 'texmode', 'on')
      | port_label('output', 1, 'x')
      | port_label('output', 2, 'y')
      | port_label('output', 3, '\theta', 'texmode', 'on')
      | port_label('output', 4, '\varpi', 'texmode', 'on')
  Quadrotor : Subsystem  mask{quad=[], x0=0, groundflag=on}
      mask prompts: quad "Quadrotor params"; x0 "Initial position"; groundflag "Ground"
      mask help: Quadrotor dynamics
      mask Help:
      | Integrate spatial velocity to update pose represented as a homogeneous
      | transformation.
      | 
      | <b>Parameters::</b>
      | 
      | q (struct)  A structure containing quadrotor dynamics
      | 
      | The elements of q are:
      | 
      |  J         Flyer rotational inertia matrix (3x3)
      |  h         Height of rotors above CoG (1x1)
      |  d         Length of flyer arms (1x1)
      |  nb        Number of blades per rotor (1x1)
      |  r         Rotor radius (1x1)
      |  c         Blade chord (1x1)
      |  e         Flapping hinge offset (1x1)
      |  Mb        Rotor blade mass (1x1)
      |  Mc        Estimated hub clamp mass (1x1)
      |  ec        Blade root clamp displacement (1x1)
      |  Ib        Rotor blade rotational inertia (1x1)
      |  Ic        Estimated root clamp inertia (1x1)
      |  mb        Static blade moment (1x1)
      |  Ir        Total rotor inertia (1x1)
      |  Ct        Non-dim. thrust coefficient (1x1)
      |  Cq        Non-dim. torque coefficient (1x1)
      |  sigma     Rotor solidity ratio (1x1)
      |  thetat    Blade tip angle (1x1)
      |  theta0    Blade root angle (1x1)
      |  theta1    Blade twist angle (1x1)
      |  theta75   3/4 blade angle (1x1)
      |  thetai    Blade ideal root approximation (1x1)
      |  a         Lift slope gradient (1x1)
      |  A         Rotor disc area (1x1)
      |  gamma     Lock number (1x1)
      | 
      | 
      | <b>Inputs::</b>
      | 
      | w1 (1x1) angular velocity of rotor 1 [rad]
      | w2 (1x1) angular velocity of rotor 2 [rad]
      | w3 (1x1) angular velocity of rotor 3 [rad]
      | w4 (1x1) angular velocity of rotor 4 [rad]
      | 
      | <b>Outputs::</b>
      | 
      | X (1x12) state vector (x, y, z, thr, thp, thy, xd, yd, zd, thrd, thpd, thyd)
      | 
      | (x,y,z) is the position in the world frame [m]
      | (thr, thp, thy) the roll/pitch/yaw orientation in the world frame [rad]
      | (xd,yd,zd) is the velocity in the body frame [m]
      | (thrd,thpd,thyd) is the roll/pitch/yaw rates in the body frame [rad/s]
      | 
      | <b>Notes::</b>
      | 
      | - See also mdl_quadrotor which defines parameters for the ANU X4 flyer.
      mask Display:
      | port_label('input',1,'\varpi','texmode','on');
      | port_label('output',1,'X','texmode','on');
  Quadrotor plot : Subsystem  mask{quad=[], xydim=2, zdim=10}
      mask prompts: quad "Model"; xydim "xy-axes dimension"; zdim "z-axis dimension"
      mask help: Animate quadrotor.
      mask Help:
      | This block graphically displays a quadrotor (flying robot).
      | 
      | A new figure is created and A graphical model of a quadrotor is animated
      | to a pose specified by the state vector input to the block.
      | 
      | The state vector is [x y z roll pitch yaw] in world coordinates and the
      | angles are in radians.
      | 
      | Notes:
      | - The dimensions of the vehicle workspace are set by parameters
  Tracking controller : Subsystem
      mask Display:
      | port_label('input', 1, 'xd^*', 'texmode', 'on')
      | port_label('input', 2, 'yd^*', 'texmode', 'on')
      | port_label('input', 3, '\theta', 'texmode', 'on')
      | port_label('output', 1, 'v', 'texmode', 'on')
      | port_label('output', 2, '\omega', 'texmode', 'on')
  Unicycle : Subsystem  mask{alim=1, vlim=1, wlim=2, x0=[0, 0, 0], a=0}
      mask prompts: alim "Acceleration"; vlim "Velocity limit"; wlim "Turn rate limit"; x0 "Initial state (x, y, theta)"; a "Coordinate frame shift (a)"
      mask help: Kino-dynamic model of unicycle vehicle, applies to differential or skid-steered vehicles.
      mask Help:
      | Kino-dynamic model of unicycle vehicle,  applies to differential or skid-steered vehicles.
      | 
      | <b>Parameters::</b>
      | 
      | Acceleration (1x1)   Vehicle acceleration limit [m/s2]
      | Velocity limit (1x1)  Vehicle speed limit [m/s]
      | Turn rate limit (1x1) Turn rate limit [rad/s]
      | Initial state (1x3) Initial state (x, y, theta)
      | Coordinate shift (1x1), moves the vehicle reference frame a distance a along the body frame x-direction.
      | 
      | <b>Inputs::</b>
      | 
      | v (1x1) velocity demand [m/s]
      | omega (1x1) rate of turn [rad/s]
      | 
      | <b>Outputs::</b>
      | 
      | x (1x1) x-coordinate in world frame [m]
      | y (1x1) x-coordinate in world frame [m]
      | theta (1x1) heading angle in world frame [rad]
      | 
      | 
      | <b>Notes::</b>
      | 
      | - Same dynamic model as the Toolbox class Vehicle.
      mask Display:
      | port_label('input', 1, 'v')
      | port_label('input', 2, '\omega', 'texmode', 'on')
      | port_label('output', 1, 'x')
      | port_label('output', 2, 'y')
      | port_label('output', 3, '\theta', 'texmode', 'on')
  vloop_voltage : Subsystem  mask{J=372e-6, B=817e-6, Km=0.228, tau_max=20, Rm=0.1, Lm=0.1, Ka=10, Kv=1, Ki=1, T=0.001}
      mask prompts: J "Inertia (K)"; B "Viscous friction coefficient (B)"; Km "Motor torque constant"; tau_max "Voltage limit (tau_max)"; Rm "Motor resistance (Rm)"; Lm "Motor inductance (Lm)"; Ka "Amplifier gain (Ka)"; Kv "Proportional gain (Kv)"; Ki "Integral gain (Ki)"; T "Sample interval (T)"
